simulink model "DC_motor_simulink"  (R2022b)
settings: Solver=VariableStepAuto  StartTime=0.0  StopTime=3  RelTol=1e-3
settings Model: Creator=Álvaro  LastModifiedBy=Álvaro

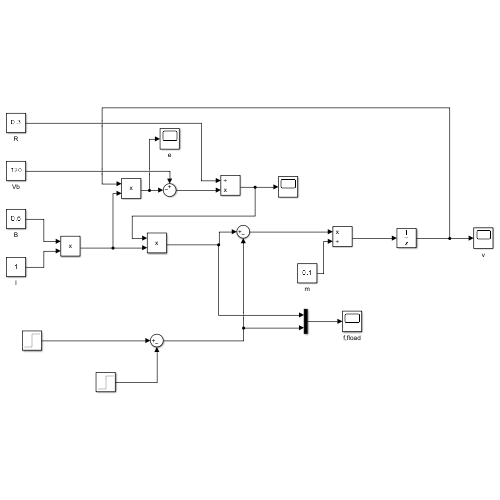
[thumbnail: Simulink's stored preview of the top-level diagram]
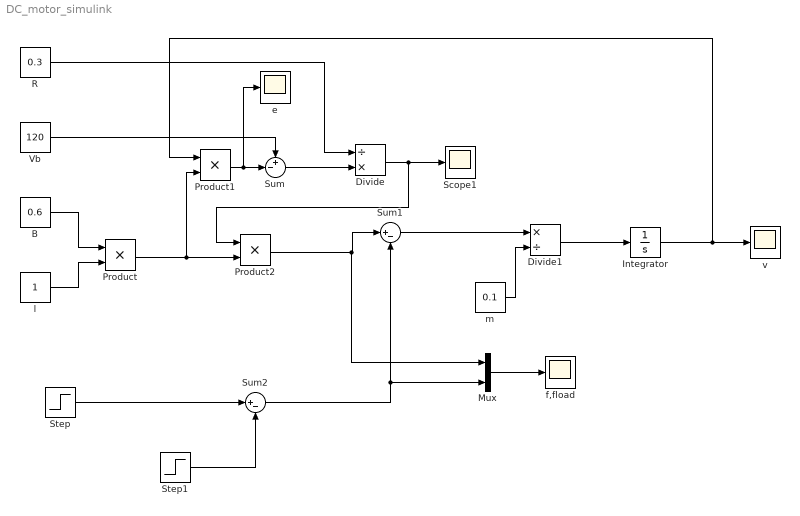
== system DC_motor_simulink ==
  B : Constant  Value=0.6
  Divide : Product  Inputs=/*
  Divide1 : Product  Inputs=*/
  Integrator : Integrator
  Mux : Mux  Inputs=2
  Product : Product
  Product1 : Product
  Product2 : Product
  R : Constant  Value=0.3
  Scope1 : Scope
  Step : Step  SampleTime=0
  Step1 : Step  SampleTime=0
  Sum : Sum  Inputs=+-|
  Sum1 : Sum  Inputs=|+-
  Sum2 : Sum  Inputs=|+-
  Vb : Constant  Value=120
  e : Scope
  f,fload : Scope
  l : Constant
  m : Constant  Value=0.1
  v : Scope
  wires:
  B/1 -> Product/1
  l/1 -> Product/2
  Vb/1 -> Sum/1
  Product1/1 -> e/1, Sum/2
  Product/1 -> Product1/2, Product2/2
  Sum/1 -> Divide/2
  R/1 -> Divide/1
  Divide/1 -> Product2/1, Scope1/1
  Product2/1 -> Mux/1, Sum1/1
  Step/1 -> Sum2/1
  Step1/1 -> Sum2/2
  Sum2/1 -> Mux/2, Sum1/2
  Sum1/1 -> Divide1/1
  m/1 -> Divide1/2
  Divide1/1 -> Integrator/1
  Integrator/1 -> Product1/1, v/1
  Mux/1 -> f,fload/1
